simulink model "r2_b16a4x512f"  (R2012b)
settings: Solver=VariableStepDiscrete  SolverMode=SingleTasking  StartTime=0.0  StopTime=1  RelTol=1e-3
undefined symbols (not defined in the file): fft_stages, n_bits_ants, n_bits_xengs
libraries: xbsIndex_r4 x27410, casper_library_misc x230, xbsReplacements_r4 x24, casper_library_delays x8, xps_library x5, casper_library_communications x4
(part 17 of 229)

== system r2_b16a4x512f/spead_time_check ==
  Constant : xbsIndex_r4/Constant  const=0  gui_display_data_type=Fixed-point  arith_type=Unsigned  n_bits=12  bin_pt=0  preci_type=Single  exp_width=8  frac_width=24  explicit_period=on  period=1  equ=P=C  opselect=C  inp2=PCIN>>17  opr=+  inp1=P  carry=CIN  dbl_ovrd=off  block_type=constant
  Constant11 : xbsIndex_r4/Constant  const=0  gui_display_data_type=Fixed-point  arith_type=Unsigned  n_bits=12  bin_pt=0  preci_type=Single  exp_width=8  frac_width=24  explicit_period=on  period=1  equ=P=C  opselect=C  inp2=PCIN>>17  opr=+  inp1=P  carry=CIN  dbl_ovrd=off  block_type=constant
  Counter : xbsIndex_r4/Counter  cnt_type=Free Running  cnt_to=Inf  operation=Up  start_count=0  cnt_by_val=1  arith_type=Unsigned  n_bits=16  bin_pt=0  load_pin=off  rst=on  en=on  explicit_period=on  period=1  dbl_ovrd=off  use_behavioral_HDL=on  implementation=Fabric  block_type=counter
  Counter1 : xbsIndex_r4/Counter  cnt_type=Free Running  cnt_to=Inf  operation=Up  start_count=0  cnt_by_val=1  arith_type=Unsigned  n_bits=16  bin_pt=0  load_pin=off  rst=on  en=on  explicit_period=on  period=1  dbl_ovrd=off  use_behavioral_HDL=on  implementation=Fabric  block_type=counter
  Delay : xbsIndex_r4/Delay  rst=off  infoeditControl=Selection of Reset will increase slice count due to use of real FFs and instead of SRLs  en=off  latency=1  dbl_ovrd=off  reg_retiming=on  block_type=delay
  Delay40 : xbsIndex_r4/Delay  rst=off  infoeditControl=Selection of Reset will increase slice count due to use of real FFs and instead of SRLs  en=off  latency=1  dbl_ovrd=off  reg_retiming=on  block_type=delay
  Delay41 : Subsystem  AncestorBlock=casper_library_delays/pipeline  mask(pipeline){latency=2}
      mask help:
      | An explicitly laid-out delay line to avoid mapping to SRL16s
      | for use in pipelining to help achieve timing closure.
      mask init:
      | pipeline_init(gcb,'latency',latency);
      settings: AttributesFormatString=Latency = %<latency>
      mask Display:
      | port_label('input', 1, 'd');
      | port_label('output', 1, 'q');
      | disp(['Z^-', num2str(latency)]);
  Delay8 : Subsystem  AncestorBlock=casper_library_delays/pipeline  mask(pipeline){latency=2}
      mask help:
      | An explicitly laid-out delay line to avoid mapping to SRL16s
      | for use in pipelining to help achieve timing closure.
      mask init:
      | pipeline_init(gcb,'latency',latency);
      settings: AttributesFormatString=Latency = %<latency>
      mask Display:
      | port_label('input', 1, 'd');
      | port_label('output', 1, 'q');
      | disp(['Z^-', num2str(latency)]);
  Delay9 : Subsystem  AncestorBlock=casper_library_delays/pipeline  mask(pipeline){latency=2}
      mask help:
      | An explicitly laid-out delay line to avoid mapping to SRL16s
      | for use in pipelining to help achieve timing closure.
      mask init:
      | pipeline_init(gcb,'latency',latency);
      settings: AttributesFormatString=Latency = %<latency>
      mask Display:
      | port_label('input', 1, 'd');
      | port_label('output', 1, 'q');
      | disp(['Z^-', num2str(latency)]);
  Logical6 : xbsIndex_r4/Logical  logical_function=AND  inputs=2  en=off  latency=0  precision=Full  arith_type=Unsigned  n_bits=16  bin_pt=0  align_bp=on  dbl_ovrd=off  block_type=logical
  Logical7 : xbsIndex_r4/Logical  logical_function=AND  inputs=2  en=off  latency=0  precision=Full  arith_type=Unsigned  n_bits=16  bin_pt=0  align_bp=on  dbl_ovrd=off  block_type=logical
  Relational : xbsIndex_r4/Relational  mode=a!=b  en=off  latency=1  dbl_ovrd=off  block_type=relational
  Relational2 : xbsIndex_r4/Relational  mode=a!=b  en=off  latency=1  dbl_ovrd=off  block_type=relational
  Slice5 : xbsIndex_r4/Slice  nbits=12  boolean_output=off  mode=Lower Bit Location + Width  bit1=0  base1=MSB of Input  bit0=0  base0=LSB of Input  dbl_ovrd=off  block_type=slice
  Slice6 : xbsIndex_r4/Slice  nbits=12  boolean_output=off  mode=Lower Bit Location + Width  bit1=0  base1=MSB of Input  bit0=0  base0=LSB of Input  dbl_ovrd=off  block_type=slice
  lsbzero0 : Outport
  lsbzero1 : Outport  Port=2
  wires:
  Delay8/1(q) -> lsbzero0/1
  Delay9/1(q) -> lsbzero1/1
  Slice5/1 -> Relational/2
  Constant/1 -> Relational/1
  Relational/1 -> Logical6/2
  Delay/1 -> Logical6/1
  Logical6/1 -> Counter/2
  [cnt_rst] -> Delay41/1(d)
  Delay41/1(q) -> Counter1/1, Counter/1
  Counter/1 -> Delay8/1(d)
  Slice6/1 -> Relational2/2
  Constant11/1 -> Relational2/1
  Relational2/1 -> Logical7/2
  Delay40/1 -> Logical7/1
  Logical7/1 -> Counter1/2
  Counter1/1 -> Delay9/1(d)
  [spead_valid0] -> Delay/1
  [spead_hdr1_0] -> Slice5/1
  [spead_valid1] -> Delay40/1
  [spead_hdr1_1] -> Slice6/1

== system r2_b16a4x512f/spead_unpack0 ==
  note: woot
  note: SPEAD header
  note: magic number - 0x53
  note: spead version
  note: item id width in bytes
  note: heap addr width in bytes
  note: <reserved>
  note: num item pointers -
      | after this header
  pkt_data : Inport
  pkt_valid : Inport  Port=2
  pkt_eof : Inport  Port=3
  Assert1 : xbsIndex_r4/Assert  assert_type=on  type_source=Explicitly  gui_display_data_type=Fixed-point  arith_type=Unsigned  n_bits=64  bin_pt=0  preci_type=Single  exp_width=8  frac_width=24  assert_rate=off  rate_source=Explicitly  period=1  output_port=on  block_type=assert
      settings: block_version=10.1.3
  Assert5 : xbsIndex_r4/Assert  assert_type=on  type_source=Explicitly  gui_display_data_type=Fixed-point  arith_type=Unsigned  n_bits=64  bin_pt=0  preci_type=Single  exp_width=8  frac_width=24  assert_rate=off  rate_source=Explicitly  period=1  output_port=on  block_type=assert
      settings: block_version=10.1.3
  Assert6 : xbsIndex_r4/Assert  assert_type=on  type_source=Explicitly  gui_display_data_type=Boolean  arith_type=Boolean  n_bits=spead_msw  bin_pt=0  preci_type=Single  exp_width=8  frac_width=24  assert_rate=off  rate_source=Explicitly  period=1  output_port=on  block_type=assert
      settings: block_version=10.1.3
  Assert7 : xbsIndex_r4/Assert  assert_type=on  type_source=Explicitly  gui_display_data_type=Boolean  arith_type=Boolean  n_bits=64  bin_pt=0  preci_type=Single  exp_width=8  frac_width=24  assert_rate=off  rate_source=Explicitly  period=1  output_port=on  block_type=assert
      settings: block_version=10.1.3
  Constant3 : xbsIndex_r4/Constant  const=83  gui_display_data_type=Fixed-point  arith_type=Unsigned  n_bits=8  bin_pt=0  preci_type=Single  exp_width=8  frac_width=24  explicit_period=on  period=1  equ=P=C  opselect=C  inp2=PCIN>>17  opr=+  inp1=P  carry=CIN  dbl_ovrd=off  block_type=constant
  Constant4 : xbsIndex_r4/Constant  const=spead_version  gui_display_data_type=Fixed-point  arith_type=Unsigned  n_bits=8  bin_pt=0  preci_type=Single  exp_width=8  frac_width=24  explicit_period=on  period=1  equ=P=C  opselect=C  inp2=PCIN>>17  opr=+  inp1=P  carry=CIN  dbl_ovrd=off  block_type=constant
  Constant7 : xbsIndex_r4/Constant  const=0  gui_display_data_type=Fixed-point  arith_type=Unsigned  n_bits=16  bin_pt=0  preci_type=Single  exp_width=8  frac_width=24  explicit_period=on  period=1  equ=P=C  opselect=C  inp2=PCIN>>17  opr=+  inp1=P  carry=CIN  dbl_ovrd=off  block_type=constant
  Delay{1..4} (4 alike) : xbsIndex_r4/Delay  rst=off  infoeditControl=Selection of Reset will increase slice count due to use of real FFs and instead of SRLs  en=off  latency=1  dbl_ovrd=off  reg_retiming=on  block_type=delay
      settings: block_version=11.4
  Inverter : xbsIndex_r4/Inverter  en=off  latency=0  dbl_ovrd=off  block_type=inv
  Logical : xbsIndex_r4/Logical  logical_function=AND  inputs=2  en=off  latency=0  precision=Full  arith_type=Unsigned  n_bits=16  bin_pt=0  align_bp=on  dbl_ovrd=off  block_type=logical
  Logical1 : xbsIndex_r4/Logical  logical_function=AND  inputs=2  en=off  latency=0  precision=Full  arith_type=Unsigned  n_bits=16  bin_pt=0  align_bp=on  dbl_ovrd=off  block_type=logical
  Logical2 : xbsIndex_r4/Logical  logical_function=AND  inputs=2  en=off  latency=0  precision=Full  arith_type=Unsigned  n_bits=16  bin_pt=0  align_bp=on  dbl_ovrd=off  block_type=logical
  Register : xbsIndex_r4/Register  init=0  rst=on  en=on  dbl_ovrd=off  block_type=register
  Relational : xbsIndex_r4/Relational  mode=a<b  en=off  latency=0  dbl_ovrd=off  block_type=relational
  badpktand : xbsIndex_r4/Logical  logical_function=AND  inputs=2  en=off  latency=0  precision=Full  arith_type=Unsigned  n_bits=16  bin_pt=0  align_bp=on  dbl_ovrd=off  block_type=logical
  check_datalen : xbsIndex_r4/Relational  mode=a!=b  en=off  latency=0  dbl_ovrd=off  block_type=relational
  data_ctr : xbsIndex_r4/Counter  cnt_type=Free Running  cnt_to=Inf  operation=Up  start_count=0  cnt_by_val=1  arith_type=Unsigned  n_bits=max_pkt_len_bits + 1  bin_pt=0  load_pin=off  rst=on  en=on  explicit_period=on  period=1  dbl_ovrd=off  use_behavioral_HDL=off  implementation=Fabric  block_type=counter
  delay : xbsIndex_r4/Delay  rst=off  infoeditControl=Selection of Reset will increase slice count due to use of real FFs and instead of SRLs  en=off  latency=2  dbl_ovrd=off  reg_retiming=on  block_type=delay
  delay1 : xbsIndex_r4/Delay  rst=off  infoeditControl=Selection of Reset will increase slice count due to use of real FFs and instead of SRLs  en=off  latency=1  dbl_ovrd=off  reg_retiming=on  block_type=delay
  delay4 : xbsIndex_r4/Delay  rst=off  infoeditControl=Selection of Reset will increase slice count due to use of real FFs and instead of SRLs  en=off  latency=2  dbl_ovrd=off  reg_retiming=on  block_type=delay
  delay5 : xbsIndex_r4/Delay  rst=off  infoeditControl=Selection of Reset will increase slice count due to use of real FFs and instead of SRLs  en=off  latency=2  dbl_ovrd=off  reg_retiming=on  block_type=delay
  delay_one : xbsIndex_r4/Delay  rst=off  infoeditControl=Selection of Reset will increase slice count due to use of real FFs and instead of SRLs  en=off  latency=1  dbl_ovrd=off  reg_retiming=on  block_type=delay
  edge_detect1 : Subsystem  AncestorBlock=casper_library_misc/edge_detect  mask(edge_detect){edge=Falling, polarity=Active High, x_in=[0 0.08 0.08 0.16 0.16 0.24 0.24 0.32 0.32 0.4], y_in=[-1 -1  1  1  1  1  1  1  1  1], x_out=[0.6 0.68 0.68 0.76 0.76 0.84 0.84 0.92 0.92 1], y_out=[-1 -1  1  1 -1 -1 -1 -1 -1 -1]}
      mask prompts: edge "Edge Type"; polarity "Output Polarity"; x_in "Input X Positions"; y_in "Input Y Positions"; x_out "Output X Positions"; y_out "Output Y Positions"
      mask help: Output is active for one-cycle after each edge of the specified type (i.e. rising, falling or both).
      mask init: same as r2_b16a4x512f/edge_detect
      settings: AttributesFormatString=|
      | falling edges
      | active high
      mask Help: Output is active for one-cycle after each edge of the specified type (i.e. rising, falling, or both).  Latency is zero.
      mask TypeOptions edge: Rising | Falling | Both
      mask TypeOptions polarity: Active High | Active Low
      mask Display:
      | plot(x_in_num,0.5+y_in_num*0.2);
      | plot(x_out_num,0.5+y_out_num*0.2);
  edge_detect2 : Subsystem  AncestorBlock=casper_library_misc/edge_detect  mask(edge_detect){edge=Falling, polarity=Active High, x_in=[0 0.08 0.08 0.16 0.16 0.24 0.24 0.32 0.32 0.4], y_in=[-1 -1  1  1  1  1  1  1  1  1], x_out=[0.6 0.68 0.68 0.76 0.76 0.84 0.84 0.92 0.92 1], y_out=[-1 -1  1  1 -1 -1 -1 -1 -1 -1]}
      mask prompts: edge "Edge Type"; polarity "Output Polarity"; x_in "Input X Positions"; y_in "Input Y Positions"; x_out "Output X Positions"; y_out "Output Y Positions"
      mask help: Output is active for one-cycle after each edge of the specified type (i.e. rising, falling or both).
      mask init: same as r2_b16a4x512f/edge_detect
      settings: AttributesFormatString=|
      | falling edges
      | active high
      mask Help: Output is active for one-cycle after each edge of the specified type (i.e. rising, falling, or both).  Latency is zero.
      mask TypeOptions edge: Rising | Falling | Both
      mask TypeOptions polarity: Active High | Active Low
      mask Display:
      | plot(x_in_num,0.5+y_in_num*0.2);
      | plot(x_out_num,0.5+y_out_num*0.2);
  edge_detect3 : Subsystem  AncestorBlock=casper_library_misc/edge_detect  mask(edge_detect){edge=Rising, polarity=Active High, x_in=[0 0.08 0.08 0.16 0.16 0.24 0.24 0.32 0.32 0.4], y_in=[-1 -1  1  1  1  1  1  1  1  1], x_out=[0.6 0.68 0.68 0.76 0.76 0.84 0.84 0.92 0.92 1], y_out=[-1 -1  1  1 -1 -1 -1 -1 -1 -1]}
      mask prompts: edge "Edge Type"; polarity "Output Polarity"; x_in "Input X Positions"; y_in "Input Y Positions"; x_out "Output X Positions"; y_out "Output Y Positions"
      mask help: Output is active for one-cycle after each edge of the specified type (i.e. rising, falling or both).
      mask init: same as r2_b16a4x512f/edge_detect
      settings: AttributesFormatString=|
      | rising edges
      | active high
      mask Help: Output is active for one-cycle after each edge of the specified type (i.e. rising, falling, or both).  Latency is zero.
      mask TypeOptions edge: Rising | Falling | Both
      mask TypeOptions polarity: Active High | Active Low
      mask Display:
      | plot(x_in_num,0.5+y_in_num*0.2);
      | plot(x_out_num,0.5+y_out_num*0.2);
  error_gate : xbsIndex_r4/Logical  logical_function=AND  inputs=2  en=off  latency=0  precision=Full  arith_type=Unsigned  n_bits=16  bin_pt=0  align_bp=on  dbl_ovrd=off  block_type=logical
  error_or : xbsIndex_r4/Logical  logical_function=OR  inputs=13  en=off  latency=0  precision=Full  arith_type=Unsigned  n_bits=16  bin_pt=0  align_bp=on  dbl_ovrd=off  block_type=logical
  hdr_chk : xbsIndex_r4/Relational  mode=a!=b  en=off  latency=1  dbl_ovrd=off  block_type=relational
  hdr_ctr : xbsIndex_r4/Counter  cnt_type=Free Running  cnt_to=Inf  operation=Up  start_count=0  cnt_by_val=1  arith_type=Unsigned  n_bits=4  bin_pt=0  load_pin=off  rst=on  en=on  explicit_period=on  period=1  dbl_ovrd=off  use_behavioral_HDL=off  implementation=Fabric  block_type=counter
  header_const1 : xbsIndex_r4/Constant  const=32769  gui_display_data_type=Fixed-point  arith_type=Unsigned  n_bits=spead_msw - spead_lsw  bin_pt=0  preci_type=Single  exp_width=8  frac_width=24  explicit_period=off  period=1  equ=P=C  opselect=C  inp2=PCIN>>17  opr=+  inp1=P  carry=CIN  dbl_ovrd=off  block_type=constant
  header_const10 : xbsIndex_r4/Constant  const=32768  gui_display_data_type=Fixed-point  arith_type=Unsigned  n_bits=spead_msw - spead_lsw  bin_pt=0  preci_type=Single  exp_width=8  frac_width=24  explicit_period=off  period=1  equ=P=C  opselect=C  inp2=PCIN>>17  opr=+  inp1=P  carry=CIN  dbl_ovrd=off  block_type=constant
  header_const11 : xbsIndex_r4/Constant  const=17152  gui_display_data_type=Fixed-point  arith_type=Unsigned  n_bits=spead_msw - spead_lsw  bin_pt=0  preci_type=Single  exp_width=8  frac_width=24  explicit_period=off  period=1  equ=P=C  opselect=C  inp2=PCIN>>17  opr=+  inp1=P  carry=CIN  dbl_ovrd=off  block_type=constant
  header_const2 : xbsIndex_r4/Constant  const=32770  gui_display_data_type=Fixed-point  arith_type=Unsigned  n_bits=spead_msw - spead_lsw  bin_pt=0  preci_type=Single  exp_width=8  frac_width=24  explicit_period=off  period=1  equ=P=C  opselect=C  inp2=PCIN>>17  opr=+  inp1=P  carry=CIN  dbl_ovrd=off  block_type=constant
  header_const3 : xbsIndex_r4/Constant  const=32771  gui_display_data_type=Fixed-point  arith_type=Unsigned  n_bits=spead_msw - spead_lsw  bin_pt=0  preci_type=Single  exp_width=8  frac_width=24  explicit_period=off  period=1  equ=P=C  opselect=C  inp2=PCIN>>17  opr=+  inp1=P  carry=CIN  dbl_ovrd=off  block_type=constant
  header_const4 : xbsIndex_r4/Constant  const=32772  gui_display_data_type=Fixed-point  arith_type=Unsigned  n_bits=spead_msw - spead_lsw  bin_pt=0  preci_type=Single  exp_width=8  frac_width=24  explicit_period=off  period=1  equ=P=C  opselect=C  inp2=PCIN>>17  opr=+  inp1=P  carry=CIN  dbl_ovrd=off  block_type=constant
  header_const5 : xbsIndex_r4/Constant  const=38400  gui_display_data_type=Fixed-point  arith_type=Unsigned  n_bits=spead_msw - spead_lsw  bin_pt=0  preci_type=Single  exp_width=8  frac_width=24  explicit_period=off  period=1  equ=P=C  opselect=C  inp2=PCIN>>17  opr=+  inp1=P  carry=CIN  dbl_ovrd=off  block_type=constant
  header_const6 : xbsIndex_r4/Constant  const=49409  gui_display_data_type=Fixed-point  arith_type=Unsigned  n_bits=spead_msw - spead_lsw  bin_pt=0  preci_type=Single  exp_width=8  frac_width=24  explicit_period=off  period=1  equ=P=C  opselect=C  inp2=PCIN>>17  opr=+  inp1=P  carry=CIN  dbl_ovrd=off  block_type=constant
  header_const7 : xbsIndex_r4/Constant  const=49411  gui_display_data_type=Fixed-point  arith_type=Unsigned  n_bits=spead_msw - spead_lsw  bin_pt=0  preci_type=Single  exp_width=8  frac_width=24  explicit_period=off  period=1  equ=P=C  opselect=C  inp2=PCIN>>17  opr=+  inp1=P  carry=CIN  dbl_ovrd=off  block_type=constant
  header_const8 : xbsIndex_r4/Constant  const=32768  gui_display_data_type=Fixed-point  arith_type=Unsigned  n_bits=spead_msw - spead_lsw  bin_pt=0  preci_type=Single  exp_width=8  frac_width=24  explicit_period=off  period=1  equ=P=C  opselect=C  inp2=PCIN>>17  opr=+  inp1=P  carry=CIN  dbl_ovrd=off  block_type=constant
  header_const9 : xbsIndex_r4/Constant  const=32768  gui_display_data_type=Fixed-point  arith_type=Unsigned  n_bits=spead_msw - spead_lsw  bin_pt=0  preci_type=Single  exp_width=8  frac_width=24  explicit_period=off  period=1  equ=P=C  opselect=C  inp2=PCIN>>17  opr=+  inp1=P  carry=CIN  dbl_ovrd=off  block_type=constant
  header_delay{1..11} (11 alike) : xbsIndex_r4/Delay  rst=off  infoeditControl=Selection of Reset will increase slice count due to use of real FFs and instead of SRLs  en=off  latency=2  dbl_ovrd=off  reg_retiming=on  block_type=delay
  header_one : xbsIndex_r4/Concat  num_inputs=6  dbl_ovrd=off  block_type=concat
      settings: block_version=10.1.3
  header_reg{1..11} (11 alike) : xbsIndex_r4/Register  init=0  rst=off  en=on  dbl_ovrd=off  block_type=register
  header_rel{1..11} (11 alike) : xbsIndex_r4/Relational  mode=a!=b  en=off  latency=1  dbl_ovrd=off  block_type=relational
  header_slice{1..11} (11 alike) : xbsIndex_r4/Slice  nbits=spead_msw - spead_lsw  boolean_output=off  mode=Upper Bit Location + Width  bit1=0  base1=MSB of Input  bit0=0  base0=LSB of Input  dbl_ovrd=off  block_type=slice
  header_vslice{1..11} (11 alike) : xbsIndex_r4/Slice  nbits=spead_lsw  boolean_output=off  mode=Lower Bit Location + Width  bit1=0  base1=MSB of Input  bit0=0  base0=LSB of Input  dbl_ovrd=off  block_type=slice
  heap_addr_width : xbsIndex_r4/Constant  const=spead_lsw/8  gui_display_data_type=Fixed-point  arith_type=Unsigned  n_bits=8  bin_pt=0  preci_type=Single  exp_width=8  frac_width=24  explicit_period=on  period=1  equ=P=C  opselect=C  inp2=PCIN>>17  opr=+  inp1=P  carry=CIN  dbl_ovrd=off  block_type=constant
  item_id_width : xbsIndex_r4/Constant  const=(spead_msw-spead_lsw)/8  gui_display_data_type=Fixed-point  arith_type=Unsigned  n_bits=8  bin_pt=0  preci_type=Single  exp_width=8  frac_width=24  explicit_period=on  period=1  equ=P=C  opselect=C  inp2=PCIN>>17  opr=+  inp1=P  carry=CIN  dbl_ovrd=off  block_type=constant
  num_headers : xbsIndex_r4/Constant  const=12  gui_display_data_type=Fixed-point  arith_type=Unsigned  n_bits=4  bin_pt=0  preci_type=Single  exp_width=8  frac_width=24  explicit_period=on  period=1  equ=P=C  opselect=C  inp2=PCIN>>17  opr=+  inp1=P  carry=CIN  dbl_ovrd=off  block_type=constant
  num_item_pts : xbsIndex_r4/Constant  const=11  gui_display_data_type=Fixed-point  arith_type=Unsigned  n_bits=16  bin_pt=0  preci_type=Single  exp_width=8  frac_width=24  explicit_period=on  period=1  equ=P=C  opselect=C  inp2=PCIN>>17  opr=+  inp1=P  carry=CIN  dbl_ovrd=off  block_type=constant
  reg_hdr_one : xbsIndex_r4/Register  init=0  rst=off  en=on  dbl_ovrd=off  block_type=register
  pkt_start : Outport
  data64 : Outport  Port=2
  valid64 : Outport  Port=3
  eof64 : Outport  Port=4
  error : Outport  Port=5
  hdr_heap_id : Outport  Port=6
  hdr_heap_size : Outport  Port=7
  hdr_heap_offset : Outport  Port=8
  hdr_pkt_len : Outport  Port=9
  hdr5_0x1600_DIR : Outport  Port=10
  hdr6_0x4101_DIR : Outport  Port=11
  hdr7_0x4103_DIR : Outport  Port=12
  hdr8_0x0000_DIR : Outport  Port=13
  hdr9_0x0000_DIR : Outport  Port=14
  hdr10_0x0000_DIR : Outport  Port=15
  hdr11_0x4300 : Outport  Port=16
  wires:
  check_datalen/1 -> badpktand/1  "160"
  delay_one/1 -> hdr_chk/1  "hdr_one"
  num_item_pts/1 -> header_one/6
  delay1/1 -> pkt_start/1  "pkt_start"
  Assert1/1 -> hdr_chk/2
  Constant7/1 -> header_one/5
  heap_addr_width/1 -> header_one/4
  item_id_width/1 -> header_one/3
  Constant4/1 -> header_one/2
  Constant3/1 -> header_one/1
  header_one/1 -> Assert1/1  "hdr_exp"
  reg_hdr_one/1 -> delay_one/1
  [hdr_word_change] -> reg_hdr_one/2
  pkt_valid/1 -> Assert7/1
  pkt_data/1 -> Assert5/1
  pkt_eof/1 -> Assert6/1
  edge_detect1/1(out) -> [gbe_start]  "gbe_start"
  Assert5/1 -> Delay4/1
  Assert7/1 -> Delay2/1
  Assert6/1 -> Delay1/1, edge_detect1/1(in)
  [gbe_start] -> Register/3, Register/1, hdr_ctr/1
  hdr_ctr/1 -> Relational/1  "hdr_ctr"
  num_headers/1 -> Relational/2
  Relational/1 -> Logical/1
  edge_detect2/1(out) -> [hdr_done]  "hdr_done"
  Register/1 -> Logical/2  "pkt_armed"
  Logical/1 -> edge_detect2/1(in), [hdr_busy]  "hdr_busy"
  [gbe_data] -> delay/1, header_reg11/1
  [hdr_busy] -> Inverter/1, data_ctr/1
  [gbe_valid] -> data_ctr/2
  data_ctr/1 -> check_datalen/1  "data_ctr"
  [gbe_eof] -> Delay3/1
  Delay3/1 -> badpktand/2
  [hdr_done] -> delay1/1  "pkt_start"
  [hdr_done] -> Register/2
  Inverter/1 -> Logical1/2
  [gbe_valid] -> Logical1/1
  edge_detect3/1(out) -> [gbe_eof]  "eof"
  [hdr_busy] -> Logical2/1
  Logical2/1 -> [hdr_word_change], hdr_ctr/2  "hdr_change"
  [gbe_valid] -> Logical2/2
  Delay1/1 -> edge_detect3/1(in)  "gbe_eof"
  Delay2/1 -> [gbe_valid]  "gbe_valid"
  Delay4/1 -> [gbe_data]  "gbe_data"
  [gbe_eof] -> delay5/1
  delay4/1 -> valid64/1  "v64"
  delay5/1 -> eof64/1, [eof_out]  "eof64"
  Logical1/1 -> delay4/1  "dv"
  delay/1 -> data64/1  "d64"
  badpktand/1 -> error_or/1
  hdr_chk/1 -> error_or/2
  error_or/1 -> error_gate/1
  [eof_out] -> error_gate/2
  error_gate/1 -> error/1
  header_reg2/1 -> header_slice2/1, header_vslice2/1, header_reg1/1
  header_reg1/1 -> header_slice1/1, header_vslice1/1, reg_hdr_one/1
  [hdr_word_change] -> header_reg1/2
  header_slice1/1 -> header_rel1/1  "spid1"
  header_vslice1/1 -> header_delay1/1
  header_const1/1 -> header_rel1/2  "exp1"
  header_delay1/1 -> hdr_heap_id/1  "hdr_heap_id"
  header_rel1/1 -> error_or/3  "err1"
  header_reg3/1 -> header_slice3/1, header_vslice3/1, header_reg2/1
  [hdr_word_change] -> header_reg2/2
  header_slice2/1 -> header_rel2/1  "spid2"
  header_vslice2/1 -> header_delay2/1
  header_const2/1 -> header_rel2/2  "exp2"
  header_delay2/1 -> hdr_heap_size/1  "hdr_heap_size"
  header_rel2/1 -> error_or/4  "err2"
  header_reg4/1 -> header_slice4/1, header_vslice4/1, header_reg3/1
  [hdr_word_change] -> header_reg3/2
  header_slice3/1 -> header_rel3/1  "spid3"
  header_vslice3/1 -> header_delay3/1
  header_const3/1 -> header_rel3/2  "exp3"
  header_delay3/1 -> hdr_heap_offset/1  "hdr_heap_offset"
  header_rel3/1 -> error_or/5  "err3"
  header_reg5/1 -> header_slice5/1, header_vslice5/1, header_reg4/1
  [hdr_word_change] -> header_reg4/2
  header_slice4/1 -> header_rel4/1  "spid4"
  header_vslice4/1 -> header_delay4/1
  header_const4/1 -> header_rel4/2  "exp4"
  header_delay4/1 -> hdr_pkt_len/1, check_datalen/2  "hdr_pkt_len"
  header_rel4/1 -> error_or/6  "err4"
  header_reg6/1 -> header_slice6/1, header_vslice6/1, header_reg5/1
  [hdr_word_change] -> header_reg5/2
  header_slice5/1 -> header_rel5/1  "spid5"
  header_vslice5/1 -> header_delay5/1
  header_const5/1 -> header_rel5/2  "exp5"
  header_delay5/1 -> hdr5_0x1600_DIR/1  "hdr5_0x1600_DIR"
  header_rel5/1 -> error_or/7  "err5"
  header_reg7/1 -> header_slice7/1, header_vslice7/1, header_reg6/1
  [hdr_word_change] -> header_reg6/2
  header_slice6/1 -> header_rel6/1  "spid6"
  header_vslice6/1 -> header_delay6/1
  header_const6/1 -> header_rel6/2  "exp6"
  header_delay6/1 -> hdr6_0x4101_DIR/1  "hdr6_0x4101_DIR"
  header_rel6/1 -> error_or/8  "err6"
  header_reg8/1 -> header_slice8/1, header_vslice8/1, header_reg7/1
  [hdr_word_change] -> header_reg7/2
  header_slice7/1 -> header_rel7/1  "spid7"
  header_vslice7/1 -> header_delay7/1
  header_const7/1 -> header_rel7/2  "exp7"
  header_delay7/1 -> hdr7_0x4103_DIR/1  "hdr7_0x4103_DIR"
  header_rel7/1 -> error_or/9  "err7"
  header_reg9/1 -> header_slice9/1, header_vslice9/1, header_reg8/1
  [hdr_word_change] -> header_reg8/2
  header_slice8/1 -> header_rel8/1  "spid8"
  header_vslice8/1 -> header_delay8/1
  header_const8/1 -> header_rel8/2  "exp8"
  header_delay8/1 -> hdr8_0x0000_DIR/1  "hdr8_0x0000_DIR"
  header_rel8/1 -> error_or/10  "err8"
  header_reg10/1 -> header_slice10/1, header_vslice10/1, header_reg9/1
  [hdr_word_change] -> header_reg9/2
  header_slice9/1 -> header_rel9/1  "spid9"
  header_vslice9/1 -> header_delay9/1
  header_const9/1 -> header_rel9/2  "exp9"
  header_delay9/1 -> hdr9_0x0000_DIR/1  "hdr9_0x0000_DIR"
  header_rel9/1 -> error_or/11  "err9"
  header_reg11/1 -> header_slice11/1, header_vslice11/1, header_reg10/1
  [hdr_word_change] -> header_reg10/2
  header_slice10/1 -> header_rel10/1  "spid10"
  header_vslice10/1 -> header_delay10/1
  header_const10/1 -> header_rel10/2  "exp10"
  header_delay10/1 -> hdr10_0x0000_DIR/1  "hdr10_0x0000_DIR"
  header_rel10/1 -> error_or/12  "err10"
  [hdr_word_change] -> header_reg11/2
  header_slice11/1 -> header_rel11/1  "spid11"
  header_vslice11/1 -> header_delay11/1
  header_const11/1 -> header_rel11/2  "exp11"
  header_delay11/1 -> hdr11_0x4300/1  "hdr11_0x4300"
  header_rel11/1 -> error_or/13  "err11"

== system r2_b16a4x512f/spead_unpack1 ==
  note: num item pointers -
      | after this header
  note: <reserved>
  note: heap addr width in bytes
  note: item id width in bytes
  note: spead version
  note: magic number - 0x53
  note: SPEAD header
  note: woot
  pkt_data : Inport
  pkt_valid : Inport  Port=2
  pkt_eof : Inport  Port=3
  Assert1 : xbsIndex_r4/Assert  assert_type=on  type_source=Explicitly  gui_display_data_type=Fixed-point  arith_type=Unsigned  n_bits=64  bin_pt=0  preci_type=Single  exp_width=8  frac_width=24  assert_rate=off  rate_source=Explicitly  period=1  output_port=on  block_type=assert
      settings: block_version=10.1.3
  Assert5 : xbsIndex_r4/Assert  assert_type=on  type_source=Explicitly  gui_display_data_type=Fixed-point  arith_type=Unsigned  n_bits=64  bin_pt=0  preci_type=Single  exp_width=8  frac_width=24  assert_rate=off  rate_source=Explicitly  period=1  output_port=on  block_type=assert
      settings: block_version=10.1.3
  Assert6 : xbsIndex_r4/Assert  assert_type=on  type_source=Explicitly  gui_display_data_type=Boolean  arith_type=Boolean  n_bits=spead_msw  bin_pt=0  preci_type=Single  exp_width=8  frac_width=24  assert_rate=off  rate_source=Explicitly  period=1  output_port=on  block_type=assert
      settings: block_version=10.1.3
  Assert7 : xbsIndex_r4/Assert  assert_type=on  type_source=Explicitly  gui_display_data_type=Boolean  arith_type=Boolean  n_bits=64  bin_pt=0  preci_type=Single  exp_width=8  frac_width=24  assert_rate=off  rate_source=Explicitly  period=1  output_port=on  block_type=assert
      settings: block_version=10.1.3
  Constant3 : xbsIndex_r4/Constant  const=83  gui_display_data_type=Fixed-point  arith_type=Unsigned  n_bits=8  bin_pt=0  preci_type=Single  exp_width=8  frac_width=24  explicit_period=on  period=1  equ=P=C  opselect=C  inp2=PCIN>>17  opr=+  inp1=P  carry=CIN  dbl_ovrd=off  block_type=constant
  Constant4 : xbsIndex_r4/Constant  const=spead_version  gui_display_data_type=Fixed-point  arith_type=Unsigned  n_bits=8  bin_pt=0  preci_type=Single  exp_width=8  frac_width=24  explicit_period=on  period=1  equ=P=C  opselect=C  inp2=PCIN>>17  opr=+  inp1=P  carry=CIN  dbl_ovrd=off  block_type=constant
  Constant7 : xbsIndex_r4/Constant  const=0  gui_display_data_type=Fixed-point  arith_type=Unsigned  n_bits=16  bin_pt=0  preci_type=Single  exp_width=8  frac_width=24  explicit_period=on  period=1  equ=P=C  opselect=C  inp2=PCIN>>17  opr=+  inp1=P  carry=CIN  dbl_ovrd=off  block_type=constant
  Delay{1..4} (4 alike) : xbsIndex_r4/Delay  rst=off  infoeditControl=Selection of Reset will increase slice count due to use of real FFs and instead of SRLs  en=off  latency=1  dbl_ovrd=off  reg_retiming=on  block_type=delay
      settings: block_version=11.4
  Inverter : xbsIndex_r4/Inverter  en=off  latency=0  dbl_ovrd=off  block_type=inv
  Logical : xbsIndex_r4/Logical  logical_function=AND  inputs=2  en=off  latency=0  precision=Full  arith_type=Unsigned  n_bits=16  bin_pt=0  align_bp=on  dbl_ovrd=off  block_type=logical
  Logical1 : xbsIndex_r4/Logical  logical_function=AND  inputs=2  en=off  latency=0  precision=Full  arith_type=Unsigned  n_bits=16  bin_pt=0  align_bp=on  dbl_ovrd=off  block_type=logical
  Logical2 : xbsIndex_r4/Logical  logical_function=AND  inputs=2  en=off  latency=0  precision=Full  arith_type=Unsigned  n_bits=16  bin_pt=0  align_bp=on  dbl_ovrd=off  block_type=logical
  Register : xbsIndex_r4/Register  init=0  rst=on  en=on  dbl_ovrd=off  block_type=register
  Relational : xbsIndex_r4/Relational  mode=a<b  en=off  latency=0  dbl_ovrd=off  block_type=relational
  badpktand : xbsIndex_r4/Logical  logical_function=AND  inputs=2  en=off  latency=0  precision=Full  arith_type=Unsigned  n_bits=16  bin_pt=0  align_bp=on  dbl_ovrd=off  block_type=logical
  check_datalen : xbsIndex_r4/Relational  mode=a!=b  en=off  latency=0  dbl_ovrd=off  block_type=relational
  data_ctr : xbsIndex_r4/Counter  cnt_type=Free Running  cnt_to=Inf  operation=Up  start_count=0  cnt_by_val=1  arith_type=Unsigned  n_bits=max_pkt_len_bits + 1  bin_pt=0  load_pin=off  rst=on  en=on  explicit_period=on  period=1  dbl_ovrd=off  use_behavioral_HDL=off  implementation=Fabric  block_type=counter
  delay : xbsIndex_r4/Delay  rst=off  infoeditControl=Selection of Reset will increase slice count due to use of real FFs and instead of SRLs  en=off  latency=2  dbl_ovrd=off  reg_retiming=on  block_type=delay
  delay1 : xbsIndex_r4/Delay  rst=off  infoeditControl=Selection of Reset will increase slice count due to use of real FFs and instead of SRLs  en=off  latency=1  dbl_ovrd=off  reg_retiming=on  block_type=delay
  delay4 : xbsIndex_r4/Delay  rst=off  infoeditControl=Selection of Reset will increase slice count due to use of real FFs and instead of SRLs  en=off  latency=2  dbl_ovrd=off  reg_retiming=on  block_type=delay
  delay5 : xbsIndex_r4/Delay  rst=off  infoeditControl=Selection of Reset will increase slice count due to use of real FFs and instead of SRLs  en=off  latency=2  dbl_ovrd=off  reg_retiming=on  block_type=delay
  delay_one : xbsIndex_r4/Delay  rst=off  infoeditControl=Selection of Reset will increase slice count due to use of real FFs and instead of SRLs  en=off  latency=1  dbl_ovrd=off  reg_retiming=on  block_type=delay
  edge_detect1 : Subsystem  AncestorBlock=casper_library_misc/edge_detect  mask(edge_detect){edge=Falling, polarity=Active High, x_in=[0 0.08 0.08 0.16 0.16 0.24 0.24 0.32 0.32 0.4], y_in=[-1 -1  1  1  1  1  1  1  1  1], x_out=[0.6 0.68 0.68 0.76 0.76 0.84 0.84 0.92 0.92 1], y_out=[-1 -1  1  1 -1 -1 -1 -1 -1 -1]}
      mask prompts: edge "Edge Type"; polarity "Output Polarity"; x_in "Input X Positions"; y_in "Input Y Positions"; x_out "Output X Positions"; y_out "Output Y Positions"
      mask help: Output is active for one-cycle after each edge of the specified type (i.e. rising, falling or both).
      mask init: same as r2_b16a4x512f/edge_detect
      settings: AttributesFormatString=|
      | falling edges
      | active high
      mask Help: Output is active for one-cycle after each edge of the specified type (i.e. rising, falling, or both).  Latency is zero.
      mask TypeOptions edge: Rising | Falling | Both
      mask TypeOptions polarity: Active High | Active Low
      mask Display:
      | plot(x_in_num,0.5+y_in_num*0.2);
      | plot(x_out_num,0.5+y_out_num*0.2);
  edge_detect2 : Subsystem  AncestorBlock=casper_library_misc/edge_detect  mask(edge_detect){edge=Falling, polarity=Active High, x_in=[0 0.08 0.08 0.16 0.16 0.24 0.24 0.32 0.32 0.4], y_in=[-1 -1  1  1  1  1  1  1  1  1], x_out=[0.6 0.68 0.68 0.76 0.76 0.84 0.84 0.92 0.92 1], y_out=[-1 -1  1  1 -1 -1 -1 -1 -1 -1]}
      mask prompts: edge "Edge Type"; polarity "Output Polarity"; x_in "Input X Positions"; y_in "Input Y Positions"; x_out "Output X Positions"; y_out "Output Y Positions"
      mask help: Output is active for one-cycle after each edge of the specified type (i.e. rising, falling or both).
      mask init: same as r2_b16a4x512f/edge_detect
      settings: AttributesFormatString=|
      | falling edges
      | active high
      mask Help: Output is active for one-cycle after each edge of the specified type (i.e. rising, falling, or both).  Latency is zero.
      mask TypeOptions edge: Rising | Falling | Both
      mask TypeOptions polarity: Active High | Active Low
      mask Display:
      | plot(x_in_num,0.5+y_in_num*0.2);
      | plot(x_out_num,0.5+y_out_num*0.2);
  edge_detect3 : Subsystem  AncestorBlock=casper_library_misc/edge_detect  mask(edge_detect){edge=Rising, polarity=Active High, x_in=[0 0.08 0.08 0.16 0.16 0.24 0.24 0.32 0.32 0.4], y_in=[-1 -1  1  1  1  1  1  1  1  1], x_out=[0.6 0.68 0.68 0.76 0.76 0.84 0.84 0.92 0.92 1], y_out=[-1 -1  1  1 -1 -1 -1 -1 -1 -1]}
      mask prompts: edge "Edge Type"; polarity "Output Polarity"; x_in "Input X Positions"; y_in "Input Y Positions"; x_out "Output X Positions"; y_out "Output Y Positions"
      mask help: Output is active for one-cycle after each edge of the specified type (i.e. rising, falling or both).
      mask init: same as r2_b16a4x512f/edge_detect
      settings: AttributesFormatString=|
      | rising edges
      | active high
      mask Help: Output is active for one-cycle after each edge of the specified type (i.e. rising, falling, or both).  Latency is zero.
      mask TypeOptions edge: Rising | Falling | Both
      mask TypeOptions polarity: Active High | Active Low
      mask Display:
      | plot(x_in_num,0.5+y_in_num*0.2);
      | plot(x_out_num,0.5+y_out_num*0.2);
  error_gate : xbsIndex_r4/Logical  logical_function=AND  inputs=2  en=off  latency=0  precision=Full  arith_type=Unsigned  n_bits=16  bin_pt=0  align_bp=on  dbl_ovrd=off  block_type=logical
  error_or : xbsIndex_r4/Logical  logical_function=OR  inputs=13  en=off  latency=0  precision=Full  arith_type=Unsigned  n_bits=16  bin_pt=0  align_bp=on  dbl_ovrd=off  block_type=logical
  hdr_chk : xbsIndex_r4/Relational  mode=a!=b  en=off  latency=1  dbl_ovrd=off  block_type=relational
  hdr_ctr : xbsIndex_r4/Counter  cnt_type=Free Running  cnt_to=Inf  operation=Up  start_count=0  cnt_by_val=1  arith_type=Unsigned  n_bits=4  bin_pt=0  load_pin=off  rst=on  en=on  explicit_period=on  period=1  dbl_ovrd=off  use_behavioral_HDL=off  implementation=Fabric  block_type=counter
  header_const1 : xbsIndex_r4/Constant  const=32769  gui_display_data_type=Fixed-point  arith_type=Unsigned  n_bits=spead_msw - spead_lsw  bin_pt=0  preci_type=Single  exp_width=8  frac_width=24  explicit_period=off  period=1  equ=P=C  opselect=C  inp2=PCIN>>17  opr=+  inp1=P  carry=CIN  dbl_ovrd=off  block_type=constant
  header_const10 : xbsIndex_r4/Constant  const=32768  gui_display_data_type=Fixed-point  arith_type=Unsigned  n_bits=spead_msw - spead_lsw  bin_pt=0  preci_type=Single  exp_width=8  frac_width=24  explicit_period=off  period=1  equ=P=C  opselect=C  inp2=PCIN>>17  opr=+  inp1=P  carry=CIN  dbl_ovrd=off  block_type=constant
  header_const11 : xbsIndex_r4/Constant  const=17152  gui_display_data_type=Fixed-point  arith_type=Unsigned  n_bits=spead_msw - spead_lsw  bin_pt=0  preci_type=Single  exp_width=8  frac_width=24  explicit_period=off  period=1  equ=P=C  opselect=C  inp2=PCIN>>17  opr=+  inp1=P  carry=CIN  dbl_ovrd=off  block_type=constant
  header_const2 : xbsIndex_r4/Constant  const=32770  gui_display_data_type=Fixed-point  arith_type=Unsigned  n_bits=spead_msw - spead_lsw  bin_pt=0  preci_type=Single  exp_width=8  frac_width=24  explicit_period=off  period=1  equ=P=C  opselect=C  inp2=PCIN>>17  opr=+  inp1=P  carry=CIN  dbl_ovrd=off  block_type=constant
  header_const3 : xbsIndex_r4/Constant  const=32771  gui_display_data_type=Fixed-point  arith_type=Unsigned  n_bits=spead_msw - spead_lsw  bin_pt=0  preci_type=Single  exp_width=8  frac_width=24  explicit_period=off  period=1  equ=P=C  opselect=C  inp2=PCIN>>17  opr=+  inp1=P  carry=CIN  dbl_ovrd=off  block_type=constant
  header_const4 : xbsIndex_r4/Constant  const=32772  gui_display_data_type=Fixed-point  arith_type=Unsigned  n_bits=spead_msw - spead_lsw  bin_pt=0  preci_type=Single  exp_width=8  frac_width=24  explicit_period=off  period=1  equ=P=C  opselect=C  inp2=PCIN>>17  opr=+  inp1=P  carry=CIN  dbl_ovrd=off  block_type=constant
  header_const5 : xbsIndex_r4/Constant  const=38400  gui_display_data_type=Fixed-point  arith_type=Unsigned  n_bits=spead_msw - spead_lsw  bin_pt=0  preci_type=Single  exp_width=8  frac_width=24  explicit_period=off  period=1  equ=P=C  opselect=C  inp2=PCIN>>17  opr=+  inp1=P  carry=CIN  dbl_ovrd=off  block_type=constant
  header_const6 : xbsIndex_r4/Constant  const=49409  gui_display_data_type=Fixed-point  arith_type=Unsigned  n_bits=spead_msw - spead_lsw  bin_pt=0  preci_type=Single  exp_width=8  frac_width=24  explicit_period=off  period=1  equ=P=C  opselect=C  inp2=PCIN>>17  opr=+  inp1=P  carry=CIN  dbl_ovrd=off  block_type=constant
  header_const7 : xbsIndex_r4/Constant  const=49411  gui_display_data_type=Fixed-point  arith_type=Unsigned  n_bits=spead_msw - spead_lsw  bin_pt=0  preci_type=Single  exp_width=8  frac_width=24  explicit_period=off  period=1  equ=P=C  opselect=C  inp2=PCIN>>17  opr=+  inp1=P  carry=CIN  dbl_ovrd=off  block_type=constant
  header_const8 : xbsIndex_r4/Constant  const=32768  gui_display_data_type=Fixed-point  arith_type=Unsigned  n_bits=spead_msw - spead_lsw  bin_pt=0  preci_type=Single  exp_width=8  frac_width=24  explicit_period=off  period=1  equ=P=C  opselect=C  inp2=PCIN>>17  opr=+  inp1=P  carry=CIN  dbl_ovrd=off  block_type=constant
  header_const9 : xbsIndex_r4/Constant  const=32768  gui_display_data_type=Fixed-point  arith_type=Unsigned  n_bits=spead_msw - spead_lsw  bin_pt=0  preci_type=Single  exp_width=8  frac_width=24  explicit_period=off  period=1  equ=P=C  opselect=C  inp2=PCIN>>17  opr=+  inp1=P  carry=CIN  dbl_ovrd=off  block_type=constant
  header_delay{1..11} (11 alike) : xbsIndex_r4/Delay  rst=off  infoeditControl=Selection of Reset will increase slice count due to use of real FFs and instead of SRLs  en=off  latency=2  dbl_ovrd=off  reg_retiming=on  block_type=delay
  header_one : xbsIndex_r4/Concat  num_inputs=6  dbl_ovrd=off  block_type=concat
      settings: block_version=10.1.3
  header_reg{1..11} (11 alike) : xbsIndex_r4/Register  init=0  rst=off  en=on  dbl_ovrd=off  block_type=register
  header_rel{1..11} (11 alike) : xbsIndex_r4/Relational  mode=a!=b  en=off  latency=1  dbl_ovrd=off  block_type=relational
  header_slice{1..11} (11 alike) : xbsIndex_r4/Slice  nbits=spead_msw - spead_lsw  boolean_output=off  mode=Upper Bit Location + Width  bit1=0  base1=MSB of Input  bit0=0  base0=LSB of Input  dbl_ovrd=off  block_type=slice
  header_vslice{1..11} (11 alike) : xbsIndex_r4/Slice  nbits=spead_lsw  boolean_output=off  mode=Lower Bit Location + Width  bit1=0  base1=MSB of Input  bit0=0  base0=LSB of Input  dbl_ovrd=off  block_type=slice
  heap_addr_width : xbsIndex_r4/Constant  const=spead_lsw/8  gui_display_data_type=Fixed-point  arith_type=Unsigned  n_bits=8  bin_pt=0  preci_type=Single  exp_width=8  frac_width=24  explicit_period=on  period=1  equ=P=C  opselect=C  inp2=PCIN>>17  opr=+  inp1=P  carry=CIN  dbl_ovrd=off  block_type=constant
  item_id_width : xbsIndex_r4/Constant  const=(spead_msw-spead_lsw)/8  gui_display_data_type=Fixed-point  arith_type=Unsigned  n_bits=8  bin_pt=0  preci_type=Single  exp_width=8  frac_width=24  explicit_period=on  period=1  equ=P=C  opselect=C  inp2=PCIN>>17  opr=+  inp1=P  carry=CIN  dbl_ovrd=off  block_type=constant
  num_headers : xbsIndex_r4/Constant  const=12  gui_display_data_type=Fixed-point  arith_type=Unsigned  n_bits=4  bin_pt=0  preci_type=Single  exp_width=8  frac_width=24  explicit_period=on  period=1  equ=P=C  opselect=C  inp2=PCIN>>17  opr=+  inp1=P  carry=CIN  dbl_ovrd=off  block_type=constant
  num_item_pts : xbsIndex_r4/Constant  const=11  gui_display_data_type=Fixed-point  arith_type=Unsigned  n_bits=16  bin_pt=0  preci_type=Single  exp_width=8  frac_width=24  explicit_period=on  period=1  equ=P=C  opselect=C  inp2=PCIN>>17  opr=+  inp1=P  carry=CIN  dbl_ovrd=off  block_type=constant
  reg_hdr_one : xbsIndex_r4/Register  init=0  rst=off  en=on  dbl_ovrd=off  block_type=register
  pkt_start : Outport
  data64 : Outport  Port=2
  valid64 : Outport  Port=3
  eof64 : Outport  Port=4
  error : Outport  Port=5
  hdr_heap_id : Outport  Port=6
  hdr_heap_size : Outport  Port=7
  hdr_heap_offset : Outport  Port=8
  hdr_pkt_len : Outport  Port=9
  hdr5_0x1600_DIR : Outport  Port=10
  hdr6_0x4101_DIR : Outport  Port=11
  hdr7_0x4103_DIR : Outport  Port=12
  hdr8_0x0000_DIR : Outport  Port=13
  hdr9_0x0000_DIR : Outport  Port=14
  hdr10_0x0000_DIR : Outport  Port=15
  hdr11_0x4300 : Outport  Port=16
  wires:
  header_rel11/1 -> error_or/13  "err11"
  header_delay11/1 -> hdr11_0x4300/1  "hdr11_0x4300"
  header_const11/1 -> header_rel11/2  "exp11"
  header_vslice11/1 -> header_delay11/1
  header_slice11/1 -> header_rel11/1  "spid11"
  [hdr_word_change] -> header_reg11/2
  header_rel10/1 -> error_or/12  "err10"
  header_delay10/1 -> hdr10_0x0000_DIR/1  "hdr10_0x0000_DIR"
  header_const10/1 -> header_rel10/2  "exp10"
  header_vslice10/1 -> header_delay10/1
  header_slice10/1 -> header_rel10/1  "spid10"
  [hdr_word_change] -> header_reg10/2
  header_reg11/1 -> header_vslice11/1, header_slice11/1, header_reg10/1
  header_rel9/1 -> error_or/11  "err9"
  header_delay9/1 -> hdr9_0x0000_DIR/1  "hdr9_0x0000_DIR"
  header_const9/1 -> header_rel9/2  "exp9"
  header_vslice9/1 -> header_delay9/1
  header_slice9/1 -> header_rel9/1  "spid9"
  [hdr_word_change] -> header_reg9/2
  header_reg10/1 -> header_vslice10/1, header_slice10/1, header_reg9/1
  header_rel8/1 -> error_or/10  "err8"
  header_delay8/1 -> hdr8_0x0000_DIR/1  "hdr8_0x0000_DIR"
  header_const8/1 -> header_rel8/2  "exp8"
  header_vslice8/1 -> header_delay8/1
  header_slice8/1 -> header_rel8/1  "spid8"
  [hdr_word_change] -> header_reg8/2
  header_reg9/1 -> header_vslice9/1, header_slice9/1, header_reg8/1
  header_rel7/1 -> error_or/9  "err7"
  header_delay7/1 -> hdr7_0x4103_DIR/1  "hdr7_0x4103_DIR"
  header_const7/1 -> header_rel7/2  "exp7"
  header_vslice7/1 -> header_delay7/1
  header_slice7/1 -> header_rel7/1  "spid7"
  [hdr_word_change] -> header_reg7/2
  header_reg8/1 -> header_vslice8/1, header_slice8/1, header_reg7/1
  header_rel6/1 -> error_or/8  "err6"
  header_delay6/1 -> hdr6_0x4101_DIR/1  "hdr6_0x4101_DIR"
  header_const6/1 -> header_rel6/2  "exp6"
  header_vslice6/1 -> header_delay6/1
  header_slice6/1 -> header_rel6/1  "spid6"
  [hdr_word_change] -> header_reg6/2
  header_reg7/1 -> header_vslice7/1, header_slice7/1, header_reg6/1
  header_rel5/1 -> error_or/7  "err5"
  header_delay5/1 -> hdr5_0x1600_DIR/1  "hdr5_0x1600_DIR"
  header_const5/1 -> header_rel5/2  "exp5"
  header_vslice5/1 -> header_delay5/1
  header_slice5/1 -> header_rel5/1  "spid5"
  [hdr_word_change] -> header_reg5/2
  header_reg6/1 -> header_vslice6/1, header_slice6/1, header_reg5/1
  header_rel4/1 -> error_or/6  "err4"
  header_delay4/1 -> check_datalen/2, hdr_pkt_len/1  "hdr_pkt_len"
  header_const4/1 -> header_rel4/2  "exp4"
  header_vslice4/1 -> header_delay4/1
  header_slice4/1 -> header_rel4/1  "spid4"
  [hdr_word_change] -> header_reg4/2
  header_reg5/1 -> header_vslice5/1, header_slice5/1, header_reg4/1
  header_rel3/1 -> error_or/5  "err3"
  header_delay3/1 -> hdr_heap_offset/1  "hdr_heap_offset"
  header_const3/1 -> header_rel3/2  "exp3"
  header_vslice3/1 -> header_delay3/1
  header_slice3/1 -> header_rel3/1  "spid3"
  [hdr_word_change] -> header_reg3/2
  header_reg4/1 -> header_vslice4/1, header_slice4/1, header_reg3/1
  header_rel2/1 -> error_or/4  "err2"
  header_delay2/1 -> hdr_heap_size/1  "hdr_heap_size"
  header_const2/1 -> header_rel2/2  "exp2"
  header_vslice2/1 -> header_delay2/1
  header_slice2/1 -> header_rel2/1  "spid2"
  [hdr_word_change] -> header_reg2/2
  header_reg3/1 -> header_vslice3/1, header_slice3/1, header_reg2/1
  header_rel1/1 -> error_or/3  "err1"
  header_delay1/1 -> hdr_heap_id/1  "hdr_heap_id"
  header_const1/1 -> header_rel1/2  "exp1"
  header_vslice1/1 -> header_delay1/1
  header_slice1/1 -> header_rel1/1  "spid1"
  [hdr_word_change] -> header_reg1/2
  header_reg1/1 -> header_vslice1/1, header_slice1/1, reg_hdr_one/1
  header_reg2/1 -> header_vslice2/1, header_slice2/1, header_reg1/1
  error_gate/1 -> error/1
  [eof_out] -> error_gate/2
  error_or/1 -> error_gate/1
  hdr_chk/1 -> error_or/2
  badpktand/1 -> error_or/1
  delay/1 -> data64/1  "d64"
  Logical1/1 -> delay4/1  "dv"
  delay5/1 -> [eof_out], eof64/1  "eof64"
  delay4/1 -> valid64/1  "v64"
  [gbe_eof] -> delay5/1
  Delay4/1 -> [gbe_data]  "gbe_data"
  Delay2/1 -> [gbe_valid]  "gbe_valid"
  Delay1/1 -> edge_detect3/1(in)  "gbe_eof"
  [gbe_valid] -> Logical2/2
  Logical2/1 -> hdr_ctr/2, [hdr_word_change]  "hdr_change"
  [hdr_busy] -> Logical2/1
  edge_detect3/1(out) -> [gbe_eof]  "eof"
  [gbe_valid] -> Logical1/1
  Inverter/1 -> Logical1/2
  [hdr_done] -> Register/2
  [hdr_done] -> delay1/1  "pkt_start"
  Delay3/1 -> badpktand/2
  [gbe_eof] -> Delay3/1
  data_ctr/1 -> check_datalen/1  "data_ctr"
  [gbe_valid] -> data_ctr/2
  [hdr_busy] -> data_ctr/1, Inverter/1
  [gbe_data] -> header_reg11/1, delay/1
  Logical/1 -> [hdr_busy], edge_detect2/1(in)  "hdr_busy"
  Register/1 -> Logical/2  "pkt_armed"
  edge_detect2/1(out) -> [hdr_done]  "hdr_done"
  Relational/1 -> Logical/1
  num_headers/1 -> Relational/2
  hdr_ctr/1 -> Relational/1  "hdr_ctr"
  [gbe_start] -> hdr_ctr/1, Register/1, Register/3
  Assert6/1 -> edge_detect1/1(in), Delay1/1
  Assert7/1 -> Delay2/1
  Assert5/1 -> Delay4/1
  edge_detect1/1(out) -> [gbe_start]  "gbe_start"
  pkt_eof/1 -> Assert6/1
  pkt_data/1 -> Assert5/1
  pkt_valid/1 -> Assert7/1
  [hdr_word_change] -> reg_hdr_one/2
  reg_hdr_one/1 -> delay_one/1
  header_one/1 -> Assert1/1  "hdr_exp"
  Constant3/1 -> header_one/1
  Constant4/1 -> header_one/2
  item_id_width/1 -> header_one/3
  heap_addr_width/1 -> header_one/4
  Constant7/1 -> header_one/5
  Assert1/1 -> hdr_chk/2
  delay1/1 -> pkt_start/1  "pkt_start"
  num_item_pts/1 -> header_one/6
  delay_one/1 -> hdr_chk/1  "hdr_one"
  check_datalen/1 -> badpktand/1  "160"
